simulink model "MMC_phase_centralized_HAAS_20260927"  (R2024b)
settings: Solver=FixedStepDiscrete  StartTime=t_init_sim  StopTime=sim_time  FixedStep=Ts  RelTol=1e-3
values from neighbouring files (symbols this model uses):
  a = 1    [script_MMC_phase_hackathon_NLM_centralized_HAAS_20260927.m]
  C1low1_active = 1    [script_MMC_phase_hackathon_NLM_centralized_HAAS_20260927.m]
  C2low1_active = 1    [script_MMC_phase_hackathon_NLM_centralized_HAAS_20260927.m]
  C_bus = 4400e-6    (= 0.0044)    [script_MMC_phase_hackathon_NLM_centralized_HAAS_20260927.m]
  C_M_extra = C_m-twist_high_side_C    [script_MMC_phase_hackathon_NLM_centralized_HAAS_20260927.m]
  duty_cycle = 1.0    (= 1)    [script_MMC_phase_hackathon_NLM_centralized_HAAS_20260927.m]
  f0 = 50    [script_MMC_phase_hackathon_NLM_centralized_HAAS_20260927.m]
  feeder_current_lower_rate_limit = -10    [script_MMC_phase_hackathon_NLM_centralized_HAAS_20260927.m]    (also in twist_parameters.m = -500)
  feeder_current_tab = [0.328 0.217 0.162 0.132 0.109 0.094 0.083 0.075 0.068 0.062 0.058 0.054 ... (42 elements, 14x3)]    [feeder_current.mat]
  feeder_current_upper_rate_limit = 0.386/(20e-3)    (= 19.3)    [twist_parameters.m]
  is6VExternallySupplied = true    [script_MMC_phase_hackathon_NLM_centralized_HAAS_20260927.m]
  isFeederJumperOpen = true    [script_MMC_phase_hackathon_NLM_centralized_HAAS_20260927.m]
  L_arm = 30e-3    (= 0.03)    [script_MMC_phase_hackathon_NLM_centralized_HAAS_20260927.m]
  m = 1    [script_MMC_phase_hackathon_NLM_centralized_HAAS_20260927.m]
  N = 5    [script_MMC_phase_hackathon_NLM_centralized_HAAS_20260927.m]
  power_losses = false    [script_MMC_phase_hackathon_NLM_centralized_HAAS_20260927.m]
  R = 15    [script_MMC_phase_hackathon_NLM_centralized_HAAS_20260927.m]
  R_arm = 0.2    [script_MMC_phase_hackathon_NLM_centralized_HAAS_20260927.m]
  source_V = 0    [script_MMC_phase_hackathon_NLM_centralized_HAAS_20260927.m]
  Tcom_sample = round(Tcom / Ts)    [script_MMC_phase_hackathon_NLM_centralized_HAAS_20260927.m]
  time_charge = 0.1    [script_MMC_phase_hackathon_NLM_centralized_HAAS_20260927.m]
  time_decharge = 1.5    [script_MMC_phase_hackathon_NLM_centralized_HAAS_20260927.m]
  Ts = 1e-6    (= 1e-06)    [script_MMC_phase_hackathon_NLM_centralized_HAAS_20260927.m]
  twist_data_acquisition_delay = 50e-9    (= 5e-08)    [script_MMC_phase_hackathon_NLM_centralized_HAAS_20260927.m]    (also in twist_parameters.m)
  twist_data_sampling_period = 1/twist_freq_data_sampling    (= 5e-05)    [script_MMC_phase_hackathon_NLM_centralized_HAAS_20260927.m]    (also in twist_parameters.m)
  twist_dead_time = 200e-9    (= 2e-07)    [twist_parameters.m]
  twist_freq_switching = 200e3    (= 200000)    [twist_parameters.m]
  twist_high_side_adc_R = 1/(1/2e6 + 1/2e6 + 1/(330e3+5.6e3))    (= 251272.836178)    [twist_parameters.m]
  twist_high_side_C = 33e-6*4 + 4.7e-6*12    (= 0.0001884)    [twist_parameters.m]
  twist_high_side_feeder_R = 47e3+4.7e3    (= 51700)    [twist_parameters.m]
  twist_high_side_rC = 0.1    [twist_parameters.m]
  twist_low_side_adc_R = 150e3+470    (= 150470)    [twist_parameters.m]
  twist_low_side_C_ceramic = 3*4.7e-6    (= 1.41e-05)    [twist_parameters.m]
  twist_low_side_C_electrolytic = 47e-6    (= 4.7e-05)    [twist_parameters.m]
  twist_low_side_L = 33e-6    (= 3.3e-05)    [twist_parameters.m]
  twist_low_side_rC = 700e-3    (= 0.7)    [twist_parameters.m]
  twist_low_side_rL = 20e-3    (= 0.02)    [twist_parameters.m]
  twist_R_VCC = (tau_VCC/twist_high_side_C  - twist_high_side_rC)/(1-(tau_VCC/twist_high_side_C - twist_high_side_rC)/R_parallel)    (= 1110.74997822)    [twist_parameters.m]
  VDC = 48    [script_MMC_phase_hackathon_NLM_centralized_HAAS_20260927.m]
undefined symbols (not defined in the file or in its folder): C_SM, feeder_current, gcbh, sps_rtmsupport, twist_low_side_lC
libraries: spsSeriesRLCBranchLib x135, spsTriangleGeneratorLib x60, spsMosfetLib x60, spsCurrentMeasurementLib x43, spsVoltageMeasurementLib x35, spsControlledCurrentSourceLib x30, spsDiodeLib x22, spsIdealSwitchLib x20, spsControlledVoltageSourceLib x1, spsGroundLib x1, spspowerguiLib x1
(part 2 of 22)

== system MMC_phase_centralized_HAAS_20260927/ /Sinus Modulation + Sorting Algorithm/M5 MCU1 ==
  g_u : Inport
  M_number : Inport  Port=2
  CVB_upper : MATLAB Function  TreatAsAtomicUnit=on
  g_unitaire_stack : Outport
  wires:
  g_u/1 -> CVB_upper/1(g)
  M_number/1 -> CVB_upper/2(M_number)
  CVB_upper/1(y) -> g_unitaire_stack/1

== system MMC_phase_centralized_HAAS_20260927/ /Sinus Modulation + Sorting Algorithm/M5 MCU2 ==
  g_u : Inport
  M_number : Inport  Port=2
  CVB_upper : MATLAB Function  TreatAsAtomicUnit=on
  g_unitaire_stack : Outport
  wires:
  g_u/1 -> CVB_upper/1(g)
  M_number/1 -> CVB_upper/2(M_number)
  CVB_upper/1(y) -> g_unitaire_stack/1

== system MMC_phase_centralized_HAAS_20260927/ /Sinus Modulation + Sorting Algorithm/M5 MCU3 ==
  g_u : Inport
  M_number : Inport  Port=2
  CVB_upper : MATLAB Function  TreatAsAtomicUnit=on
  g_unitaire_stack : Outport
  wires:
  g_u/1 -> CVB_upper/1(g)
  M_number/1 -> CVB_upper/2(M_number)
  CVB_upper/1(y) -> g_unitaire_stack/1

== system MMC_phase_centralized_HAAS_20260927/ /Sinus Modulation + Sorting Algorithm/M5 MCU4 ==
  g_u : Inport
  M_number : Inport  Port=2
  CVB_upper : MATLAB Function  TreatAsAtomicUnit=on
  g_unitaire_stack : Outport
  wires:
  g_u/1 -> CVB_upper/1(g)
  M_number/1 -> CVB_upper/2(M_number)
  CVB_upper/1(y) -> g_unitaire_stack/1

== system MMC_phase_centralized_HAAS_20260927/ /Sinus Modulation + Sorting Algorithm/M5 MCU5 ==
  g_u : Inport
  M_number : Inport  Port=2
  CVB_upper : MATLAB Function  TreatAsAtomicUnit=on
  g_unitaire_stack : Outport
  wires:
  g_u/1 -> CVB_upper/1(g)
  M_number/1 -> CVB_upper/2(M_number)
  CVB_upper/1(y) -> g_unitaire_stack/1

== system MMC_phase_centralized_HAAS_20260927/ /Sinus Modulation + Sorting Algorithm/Supervisor MCU ==
  note: NLM
  note: NLM
  note: Modulation reference
  note: Sorting and CVB algorithm - Upper and Lower stacks
  note: NLM modulation
  Vc_U : Inport
  I_U : Inport  Port=2
  Vc_L : Inport  Port=3
  I_L : Inport  Port=4
  Constant : Constant
  Constant1 : Constant  Value=0
  Constant2 : Constant
  Constant3 : Constant  Value=0
  Constant4 : Constant  Value=a*1/2
  Gain : Gain  Gain=N
  Gain1 : Gain  Gain=m*1/2
  Gain2 : Gain  Gain=N
  GreaterThan : RelationalOperator  Operator=~=  OutDataTypeStr=boolean  RndMeth=Simplest  InputSameDT=off
  GreaterThan1 : RelationalOperator  Operator=~=  OutDataTypeStr=boolean  RndMeth=Simplest  InputSameDT=off
  Memory : Memory  InheritSampleTime=on  LinearizeMemory=on  LinearizeAsDelay=on
  Memory1 : Memory  InheritSampleTime=on  LinearizeMemory=on  LinearizeAsDelay=on
  Quantizer : Quantizer  QuantizationInterval=1
  Quantizer1 : Quantizer  QuantizationInterval=1
  Saturation : Saturate  UpperLimit=N  LowerLimit=0
  Saturation1 : Saturate  UpperLimit=N  LowerLimit=0
  Sine Wave : Sin  Frequency=2*pi*f0  SampleTime=Ts
  Sorting_CVB_Lower : Subsystem
      settings: PortSchema="{\"entries\":[{\"content\":{\"sides\":[{\"content\":{\"connectorIds\":[\"In1\",\"In2\",\"In3\"]},\"type\":\"ConnectorPlacement.EquallySpacedRectSide\",\"uuid\":\"25566ff9-210a-4488-8b15-702d65e93a4b\"},{\"content\":{\"connectorIds\":[\"Out1\"],\"side\":\"RIGHT\"},\"type\":\"ConnectorPlacement.EquallySpacedRectSide\",\"uuid\":\"97373fc2-3782-4e65-8804-644d53fa5380\"},{\"content\":{\"connectorIds\":[\"In4\"],\"side\":\"TOP\"},\"type\":\"ConnectorPlacement.EquallySpacedRectSide\",\"uuid\":\"e65d2433-d029-4e4a-b081-22e9ded4f272\"}]},\"type\":\"ConnectorPlacement.EquallySpacedConnector\",\"uuid\":\"235c80e7-78ad-4e69-a231-ec76d675b4ae\"}],\"packageUris\":[\"http://schema.mathworks.com/mf0/Connector/R2020b\"],\"version\":\"1.0\"}"
  Sorting_CVB_Upper : Subsystem
      settings: PortSchema="{\"entries\":[{\"content\":{\"sides\":[{\"content\":{\"connectorIds\":[\"In1\",\"In2\",\"In3\"]},\"type\":\"ConnectorPlacement.EquallySpacedRectSide\",\"uuid\":\"25566ff9-210a-4488-8b15-702d65e93a4b\"},{\"content\":{\"connectorIds\":[\"Out1\"],\"side\":\"RIGHT\"},\"type\":\"ConnectorPlacement.EquallySpacedRectSide\",\"uuid\":\"97373fc2-3782-4e65-8804-644d53fa5380\"},{\"content\":{\"connectorIds\":[\"In4\"],\"side\":\"TOP\"},\"type\":\"ConnectorPlacement.EquallySpacedRectSide\",\"uuid\":\"e65d2433-d029-4e4a-b081-22e9ded4f272\"}]},\"type\":\"ConnectorPlacement.EquallySpacedConnector\",\"uuid\":\"235c80e7-78ad-4e69-a231-ec76d675b4ae\"}],\"packageUris\":[\"http://schema.mathworks.com/mf0/Connector/R2020b\"],\"version\":\"1.0\"}"
  Sum1 : Sum  Inputs=|+-
  Sum2 : Sum  Inputs=|++
  Switch : Switch  Criteria=u2 > Threshold  SaturateOnIntegerOverflow=off  InputSameDT=off
  Switch1 : Switch  Criteria=u2 > Threshold  SaturateOnIntegerOverflow=off  InputSameDT=off
  gU : Outport
  gL : Outport  Port=2
  tag scope: N_l=global, N_u=global, ml=global, mu=global
  wires:
  Switch/1 -> Sorting_CVB_Upper/4(Pulse)
  Sorting_CVB_Lower/1(g_unitaire_stack) -> gL/1
  Vc_U/1 -> Sorting_CVB_Upper/1(Vc_unitaire_stack)
  Switch1/1 -> Sorting_CVB_Lower/4(Pulse)
  I_U/1 -> Sorting_CVB_Upper/2(i_stack)
  Quantizer1/1 -> Saturation1/1
  Sorting_CVB_Upper/1(g_unitaire_stack) -> gU/1
  Constant/1 -> Switch/1
  Sine Wave/1 -> Gain1/1
  Saturation/1 -> Sorting_CVB_Upper/3(N_on_stack), Memory/1, GreaterThan/1, [N_u]
  Constant1/1 -> Switch/3
  Saturation1/1 -> Memory1/1, GreaterThan1/1, Sorting_CVB_Lower/3(N_on_stack), [N_l]
  Gain2/1 -> Quantizer1/1
  Constant2/1 -> Switch1/1
  Quantizer/1 -> Saturation/1
  Gain/1 -> Quantizer/1
  GreaterThan/1 -> Switch/2
  Sum1/1 -> Gain/1, [mu]
  Memory1/1 -> GreaterThan1/2
  Gain1/1 -> Sum1/2, Sum2/2
  Constant3/1 -> Switch1/3
  Vc_L/1 -> Sorting_CVB_Lower/1(Vc_unitaire_stack)
  Sum2/1 -> [ml], Gain2/1
  GreaterThan1/1 -> Switch1/2
  Constant4/1 -> Sum2/1, Sum1/1
  Memory/1 -> GreaterThan/2
  I_L/1 -> Sorting_CVB_Lower/2(i_stack)

== system MMC_phase_centralized_HAAS_20260927/ /Subsystem/Subsystem ==
  note: MMC electrical circuit connected to the modules hardware block
  note: MMC electrical circuit connected to the modules hardware block
  note: MMC electrical circuit connected to the modules hardware block
  note: MMC electrical circuit connected to the modules hardware block
  note: MMC electrical circuit connected to the modules hardware block
  duty_cycle_M1 : Inport
  block_M1 : Inport  Port=2
  duty_cycle_M2 : Inport  Port=3
  block_M2 : Inport  Port=4
  duty_cycle_M3 : Inport  Port=5
  block_M3 : Inport  Port=6
  duty_cycle_M4 : Inport  Port=7
  block_M4 : Inport  Port=8
  duty_cycle_M5 : Inport  Port=9
  block_M5 : Inport  Port=10
  AC Load{6..10} (5 alike) : spsSeriesRLCBranchLib/Series RLC Branch  LConnTagsString=__new0  RConnTagsString=__new0  BranchType=C  Resistance=R  Inductance=L_arm  SetiL0=off  InitialCurrent=0  Capacitance=C_M_extra  Setx0=on  InitialVoltage=source_V  Measurements=None
  Hardware M1 : Subsystem
  Hardware M2 : Subsystem
  Hardware M3 : Subsystem
  Hardware M4 : Subsystem
  Hardware M5 : Subsystem
  V1low_M1 : PMIOPort  Side=Left
  Low_GND_M5 : PMIOPort  Port=2  Side=Left
  i_mod_M1 : Outport
  v_cap_M1 : Outport  Port=2
  v_cap_M2 : Outport  Port=3
  v_cap_M3 : Outport  Port=4
  v_cap_M4 : Outport  Port=5
  v_cap_M5 : Outport  Port=6
  wires:
  Hardware M1/1(v_cap) -> v_cap_M1/1
  duty_cycle_M1/1 -> Hardware M1/1(duty_cycle)
  duty_cycle_M2/1 -> Hardware M2/1(duty_cycle)
  block_M5/1 -> Hardware M5/2(block)
  Hardware M3/1(v_cap) -> v_cap_M3/1
  block_M1/1 -> Hardware M1/2(block)
  Hardware M1/2(i_mod) -> i_mod_M1/1
  duty_cycle_M4/1 -> Hardware M4/1(duty_cycle)
  block_M2/1 -> Hardware M2/2(block)
  Hardware M5/1(v_cap) -> v_cap_M5/1
  Hardware M2/1(v_cap) -> v_cap_M2/1
  duty_cycle_M3/1 -> Hardware M3/1(duty_cycle)
  duty_cycle_M5/1 -> Hardware M5/1(duty_cycle)
  block_M4/1 -> Hardware M4/2(block)
  block_M3/1 -> Hardware M3/2(block)
  Hardware M4/1(v_cap) -> v_cap_M4/1
  connections:
  Hardware M5/RConn2 -- AC Load10/RConn1
  AC Load6/LConn1 -- Hardware M1/RConn1
  Hardware M1/LConn2 -- Hardware M2/LConn1
  Hardware M3/LConn2 -- Hardware M4/LConn1
  Hardware M5/RConn1 -- AC Load10/LConn1
  AC Load6/RConn1 -- Hardware M1/RConn2
  Hardware M2/RConn2 -- AC Load7/RConn1
  Hardware M2/LConn2 -- Hardware M3/LConn1
  Hardware M2/RConn1 -- AC Load7/LConn1
  Hardware M3/RConn1 -- AC Load8/LConn1
  Hardware M3/RConn2 -- AC Load8/RConn1
  Hardware M4/RConn2 -- AC Load9/RConn1
  Hardware M4/RConn1 -- AC Load9/LConn1
  Hardware M4/LConn2 -- Hardware M5/LConn1
  V1low_M1/RConn1 -- Hardware M1/LConn1
  Low_GND_M5/RConn1 -- Hardware M5/LConn2

== system MMC_phase_centralized_HAAS_20260927/ /Subsystem/Subsystem1 ==
  note: MMC electrical circuit connected to the modules hardware block
  note: MMC electrical circuit connected to the modules hardware block
  note: MMC electrical circuit connected to the modules hardware block
  note: MMC electrical circuit connected to the modules hardware block
  note: MMC electrical circuit connected to the modules hardware block
  duty_cycle_M1 : Inport
  block_M1 : Inport  Port=2
  duty_cycle_M2 : Inport  Port=3
  block_M2 : Inport  Port=4
  duty_cycle_M3 : Inport  Port=5
  block_M3 : Inport  Port=6
  duty_cycle_M4 : Inport  Port=7
  block_M4 : Inport  Port=8
  duty_cycle_M5 : Inport  Port=9
  block_M5 : Inport  Port=10
  AC Load{6..10} (5 alike) : spsSeriesRLCBranchLib/Series RLC Branch  LConnTagsString=__new0  RConnTagsString=__new0  BranchType=C  Resistance=R  Inductance=L_arm  SetiL0=off  InitialCurrent=0  Capacitance=C_M_extra  Setx0=on  InitialVoltage=source_V  Measurements=None
  Hardware M1 : Subsystem
  Hardware M2 : Subsystem
  Hardware M3 : Subsystem
  Hardware M4 : Subsystem
  Hardware M5 : Subsystem
  V1low_M1 : PMIOPort  Side=Left
  Low_GND_M5 : PMIOPort  Port=2  Side=Left
  i_mod_M1 : Outport
  v_cap_M1 : Outport  Port=2
  v_cap_M2 : Outport  Port=3
  v_cap_M3 : Outport  Port=4
  v_cap_M4 : Outport  Port=5
  v_cap_M5 : Outport  Port=6
  wires:
  Hardware M1/1(v_cap) -> v_cap_M1/1
  duty_cycle_M1/1 -> Hardware M1/1(duty_cycle)
  duty_cycle_M2/1 -> Hardware M2/1(duty_cycle)
  block_M5/1 -> Hardware M5/2(block)
  Hardware M3/1(v_cap) -> v_cap_M3/1
  block_M1/1 -> Hardware M1/2(block)
  Hardware M1/2(i_mod) -> i_mod_M1/1
  duty_cycle_M4/1 -> Hardware M4/1(duty_cycle)
  block_M2/1 -> Hardware M2/2(block)
  Hardware M5/1(v_cap) -> v_cap_M5/1
  Hardware M2/1(v_cap) -> v_cap_M2/1
  duty_cycle_M3/1 -> Hardware M3/1(duty_cycle)
  duty_cycle_M5/1 -> Hardware M5/1(duty_cycle)
  block_M4/1 -> Hardware M4/2(block)
  block_M3/1 -> Hardware M3/2(block)
  Hardware M4/1(v_cap) -> v_cap_M4/1
  connections:
  Hardware M5/RConn2 -- AC Load10/RConn1
  AC Load6/LConn1 -- Hardware M1/RConn1
  Hardware M1/LConn2 -- Hardware M2/LConn1
  Hardware M3/LConn2 -- Hardware M4/LConn1
  Hardware M5/RConn1 -- AC Load10/LConn1
  AC Load6/RConn1 -- Hardware M1/RConn2
  Hardware M2/RConn2 -- AC Load7/RConn1
  Hardware M2/LConn2 -- Hardware M3/LConn1
  Hardware M2/RConn1 -- AC Load7/LConn1
  Hardware M3/RConn1 -- AC Load8/LConn1
  Hardware M3/RConn2 -- AC Load8/RConn1
  Hardware M4/RConn2 -- AC Load9/RConn1
  Hardware M4/RConn1 -- AC Load9/LConn1
  Hardware M4/LConn2 -- Hardware M5/LConn1
  V1low_M1/RConn1 -- Hardware M1/LConn1
  Low_GND_M5/RConn1 -- Hardware M5/LConn2

== system MMC_phase_centralized_HAAS_20260927/ /Communication_subsystem/Lower_arm/M1_Comm ==
  TX_variables : Inport
  sync : Inport  Port=2
  RX_signal : Inport  Port=3
  Data Type Conversion : DataTypeConversion  OutDataTypeStr=single  SaturateOnIntegerOverflow=off  RndMeth=Floor
  Delay : Delay  DelayLength=Tcom_sample
  Snapshot : MATLAB Function  TreatAsAtomicUnit=on
  TxFormatter : MATLAB Function  TreatAsAtomicUnit=on
  node_id : Constant  Value=6
  TX_signal : Outport
  RX_Variables : Outport  Port=2
  wires:
  TX_variables/1 -> Data Type Conversion/1
  RX_signal/1 -> Snapshot/1(rx_signal), TxFormatter/3(rx_signal)
  TxFormatter/1(tx_data) -> Delay/1
  Data Type Conversion/1 -> TxFormatter/1(tx_variables)
  Snapshot/1(rx_variables) -> RX_Variables/1
  sync/1 -> Snapshot/3(sync), TxFormatter/2(sync)
  node_id/1 -> TxFormatter/4(node_id)
  Delay/1 -> TX_signal/1

== system MMC_phase_centralized_HAAS_20260927/ /Communication_subsystem/Lower_arm/M2_Comm ==
  TX_variables : Inport
  sync : Inport  Port=2
  RX_signal : Inport  Port=3
  Data Type Conversion : DataTypeConversion  OutDataTypeStr=single  SaturateOnIntegerOverflow=off  RndMeth=Floor
  Delay : Delay  DelayLength=Tcom_sample
  Snapshot : MATLAB Function  TreatAsAtomicUnit=on
  TxFormatter : MATLAB Function  TreatAsAtomicUnit=on
  node_id : Constant  Value=7
  TX_signal : Outport
  RX_Variables : Outport  Port=2
  wires:
  TX_variables/1 -> Data Type Conversion/1
  RX_signal/1 -> Snapshot/1(rx_signal), TxFormatter/3(rx_signal)
  TxFormatter/1(tx_data) -> Delay/1
  Data Type Conversion/1 -> TxFormatter/1(tx_variables)
  Snapshot/1(rx_variables) -> RX_Variables/1
  sync/1 -> Snapshot/3(sync), TxFormatter/2(sync)
  node_id/1 -> TxFormatter/4(node_id)
  Delay/1 -> TX_signal/1

== system MMC_phase_centralized_HAAS_20260927/ /Communication_subsystem/Lower_arm/M3_Comm ==
  TX_variables : Inport
  sync : Inport  Port=2
  RX_signal : Inport  Port=3
  Data Type Conversion : DataTypeConversion  OutDataTypeStr=single  SaturateOnIntegerOverflow=off  RndMeth=Floor
  Delay : Delay  DelayLength=Tcom_sample
  Snapshot : MATLAB Function  TreatAsAtomicUnit=on
  TxFormatter : MATLAB Function  TreatAsAtomicUnit=on
  node_id : Constant  Value=8
  TX_signal : Outport
  RX_Variables : Outport  Port=2
  wires:
  TX_variables/1 -> Data Type Conversion/1
  RX_signal/1 -> Snapshot/1(rx_signal), TxFormatter/3(rx_signal)
  TxFormatter/1(tx_data) -> Delay/1
  Data Type Conversion/1 -> TxFormatter/1(tx_variables)
  Snapshot/1(rx_variables) -> RX_Variables/1
  sync/1 -> Snapshot/3(sync), TxFormatter/2(sync)
  node_id/1 -> TxFormatter/4(node_id)
  Delay/1 -> TX_signal/1

== system MMC_phase_centralized_HAAS_20260927/ /Communication_subsystem/Lower_arm/M4_Comm ==
  TX_variables : Inport
  sync : Inport  Port=2
  RX_signal : Inport  Port=3
  Data Type Conversion : DataTypeConversion  OutDataTypeStr=single  SaturateOnIntegerOverflow=off  RndMeth=Floor
  Delay : Delay  DelayLength=Tcom_sample
  Snapshot : MATLAB Function  TreatAsAtomicUnit=on
  TxFormatter : MATLAB Function  TreatAsAtomicUnit=on
  node_id : Constant  Value=9
  TX_signal : Outport
  RX_Variables : Outport  Port=2
  wires:
  TX_variables/1 -> Data Type Conversion/1
  RX_signal/1 -> Snapshot/1(rx_signal), TxFormatter/3(rx_signal)
  TxFormatter/1(tx_data) -> Delay/1
  Data Type Conversion/1 -> TxFormatter/1(tx_variables)
  Snapshot/1(rx_variables) -> RX_Variables/1
  sync/1 -> Snapshot/3(sync), TxFormatter/2(sync)
  node_id/1 -> TxFormatter/4(node_id)
  Delay/1 -> TX_signal/1

== system MMC_phase_centralized_HAAS_20260927/ /Communication_subsystem/Lower_arm/M5_Comm ==
  TX_variables : Inport
  sync : Inport  Port=2
  RX_signal : Inport  Port=3
  Data Type Conversion : DataTypeConversion  OutDataTypeStr=single  SaturateOnIntegerOverflow=off  RndMeth=Floor
  Delay : Delay  DelayLength=Tcom_sample
  Snapshot : MATLAB Function  TreatAsAtomicUnit=on
  TxFormatter : MATLAB Function  TreatAsAtomicUnit=on
  node_id : Constant  Value=10
  TX_signal : Outport
  RX_Variables : Outport  Port=2
  wires:
  TX_variables/1 -> Data Type Conversion/1
  RX_signal/1 -> Snapshot/1(rx_signal), TxFormatter/3(rx_signal)
  TxFormatter/1(tx_data) -> Delay/1
  Data Type Conversion/1 -> TxFormatter/1(tx_variables)
  Snapshot/1(rx_variables) -> RX_Variables/1
  sync/1 -> Snapshot/3(sync), TxFormatter/2(sync)
  node_id/1 -> TxFormatter/4(node_id)
  Delay/1 -> TX_signal/1

== system MMC_phase_centralized_HAAS_20260927/ /Communication_subsystem/Upper_arm/M1_Comm ==
  TX_variables : Inport
  sync : Inport  Port=2
  RX_signal : Inport  Port=3
  Data Type Conversion : DataTypeConversion  OutDataTypeStr=single  SaturateOnIntegerOverflow=off  RndMeth=Floor
  Delay : Delay  DelayLength=Tcom_sample
  Delay1 : Delay  DelayLength=1
  Delay2 : Delay  DelayLength=1
  Scope : Scope  NumInputPorts=6
  Scope1 : Scope  NumInputPorts=2
  Snapshot : MATLAB Function  TreatAsAtomicUnit=on
  TxFormatter : MATLAB Function  TreatAsAtomicUnit=on
  node_id : Constant
  TX_signal : Outport
  RX_Variables : Outport  Port=2
  wires:
  TX_variables/1 -> Data Type Conversion/1
  TxFormatter/1(tx_data) -> Delay/1
  Delay/1 -> TX_signal/1
  sync/1 -> Snapshot/3(sync), Scope1/1, TxFormatter/2(sync)  "Ctrl_task"
  RX_signal/1 -> Snapshot/1(rx_signal), TxFormatter/3(rx_signal)
  Snapshot/1(rx_variables) -> RX_Variables/1
  Data Type Conversion/1 -> TxFormatter/1(tx_variables)
  node_id/1 -> TxFormatter/4(node_id)
  TxFormatter/2(tx_fire) -> Scope/1
  TxFormatter/3(tx_busy) -> Scope/2
  TxFormatter/5(rx_count_dbg) -> Scope/4
  TxFormatter/6(rx_id_dbg) -> Scope1/2, Scope/5  "1 -> 2 data"
  TxFormatter/7(overrun) -> Scope/6
  TxFormatter/8(local_frame_snapshot) -> Delay1/1
  Delay1/1 -> Snapshot/2(local_frame_snapshot)
  TxFormatter/4(round_done) -> Scope/3, Delay2/1
  Delay2/1 -> Snapshot/4(round_done)

== system MMC_phase_centralized_HAAS_20260927/ /Communication_subsystem/Upper_arm/M2_Comm ==
  TX_variables : Inport
  sync : Inport  Port=2
  RX_signal : Inport  Port=3
  Data Type Conversion : DataTypeConversion  OutDataTypeStr=single  SaturateOnIntegerOverflow=off  RndMeth=Floor
  Delay : Delay  DelayLength=Tcom_sample
  Delay1 : Delay  DelayLength=1
  Scope : Scope  NumInputPorts=6
  Snapshot : MATLAB Function  TreatAsAtomicUnit=on
  TxFormatter : MATLAB Function  TreatAsAtomicUnit=on
  node_id : Constant  Value=2
  TX_signal : Outport
  RX_Variables : Outport  Port=2
  wires:
  TxFormatter/2(tx_fire) -> Scope/1
  TxFormatter/3(tx_busy) -> Scope/2
  TxFormatter/8(local_frame_snapshot) -> Delay1/1
  TxFormatter/7(overrun) -> Scope/6
  TX_variables/1 -> Data Type Conversion/1
  Delay/1 -> TX_signal/1
  TxFormatter/4(round_done) -> Scope/3
  Snapshot/1(rx_variables) -> RX_Variables/1
  TxFormatter/1(tx_data) -> Delay/1
  Delay1/1 -> Snapshot/2(local_frame_snapshot)
  Data Type Conversion/1 -> TxFormatter/1(tx_variables)
  sync/1 -> Snapshot/3(sync), TxFormatter/2(sync)
  node_id/1 -> TxFormatter/4(node_id)
  TxFormatter/6(rx_id_dbg) -> Scope/5
  RX_signal/1 -> Snapshot/1(rx_signal), TxFormatter/3(rx_signal)
  TxFormatter/5(rx_count_dbg) -> Scope/4

== system MMC_phase_centralized_HAAS_20260927/ /Communication_subsystem/Upper_arm/M3_Comm ==
  TX_variables : Inport
  sync : Inport  Port=2
  RX_signal : Inport  Port=3
  Data Type Conversion : DataTypeConversion  OutDataTypeStr=single  SaturateOnIntegerOverflow=off  RndMeth=Floor
  Delay : Delay  DelayLength=Tcom_sample
  Delay1 : Delay  DelayLength=1
  Scope : Scope  NumInputPorts=6
  Snapshot : MATLAB Function  TreatAsAtomicUnit=on
  TxFormatter : MATLAB Function  TreatAsAtomicUnit=on
  node_id : Constant  Value=3
  TX_signal : Outport
  RX_Variables : Outport  Port=2
  wires:
  TxFormatter/2(tx_fire) -> Scope/1
  TxFormatter/3(tx_busy) -> Scope/2
  TxFormatter/8(local_frame_snapshot) -> Delay1/1
  TxFormatter/7(overrun) -> Scope/6
  TX_variables/1 -> Data Type Conversion/1
  Delay/1 -> TX_signal/1
  TxFormatter/4(round_done) -> Scope/3
  Snapshot/1(rx_variables) -> RX_Variables/1
  TxFormatter/1(tx_data) -> Delay/1
  Delay1/1 -> Snapshot/2(local_frame_snapshot)
  Data Type Conversion/1 -> TxFormatter/1(tx_variables)
  sync/1 -> Snapshot/3(sync), TxFormatter/2(sync)
  node_id/1 -> TxFormatter/4(node_id)
  TxFormatter/6(rx_id_dbg) -> Scope/5
  RX_signal/1 -> Snapshot/1(rx_signal), TxFormatter/3(rx_signal)
  TxFormatter/5(rx_count_dbg) -> Scope/4

== system MMC_phase_centralized_HAAS_20260927/ /Communication_subsystem/Upper_arm/M4_Comm ==
  TX_variables : Inport
  sync : Inport  Port=2
  RX_signal : Inport  Port=3
  Data Type Conversion : DataTypeConversion  OutDataTypeStr=single  SaturateOnIntegerOverflow=off  RndMeth=Floor
  Delay : Delay  DelayLength=Tcom_sample
  Delay1 : Delay  DelayLength=1
  Scope : Scope  NumInputPorts=6
  Snapshot : MATLAB Function  TreatAsAtomicUnit=on
  TxFormatter : MATLAB Function  TreatAsAtomicUnit=on
  node_id : Constant  Value=4
  TX_signal : Outport
  RX_Variables : Outport  Port=2
  wires:
  TxFormatter/2(tx_fire) -> Scope/1
  TxFormatter/3(tx_busy) -> Scope/2
  TxFormatter/8(local_frame_snapshot) -> Delay1/1
  TxFormatter/7(overrun) -> Scope/6
  TX_variables/1 -> Data Type Conversion/1
  Delay/1 -> TX_signal/1
  TxFormatter/4(round_done) -> Scope/3
  Snapshot/1(rx_variables) -> RX_Variables/1
  TxFormatter/1(tx_data) -> Delay/1
  Delay1/1 -> Snapshot/2(local_frame_snapshot)
  Data Type Conversion/1 -> TxFormatter/1(tx_variables)
  sync/1 -> Snapshot/3(sync), TxFormatter/2(sync)
  node_id/1 -> TxFormatter/4(node_id)
  TxFormatter/6(rx_id_dbg) -> Scope/5
  RX_signal/1 -> Snapshot/1(rx_signal), TxFormatter/3(rx_signal)
  TxFormatter/5(rx_count_dbg) -> Scope/4

== system MMC_phase_centralized_HAAS_20260927/ /Communication_subsystem/Upper_arm/M5_Comm ==
  TX_variables : Inport
  sync : Inport  Port=2
  RX_signal : Inport  Port=3
  Data Type Conversion : DataTypeConversion  OutDataTypeStr=single  SaturateOnIntegerOverflow=off  RndMeth=Floor
  Delay : Delay  DelayLength=Tcom_sample
  Snapshot : MATLAB Function  TreatAsAtomicUnit=on
  TxFormatter : MATLAB Function  TreatAsAtomicUnit=on
  node_id : Constant  Value=5
  TX_signal : Outport
  RX_Variables : Outport  Port=2
  wires:
  TX_variables/1 -> Data Type Conversion/1
  RX_signal/1 -> Snapshot/1(rx_signal), TxFormatter/3(rx_signal)
  TxFormatter/1(tx_data) -> Delay/1
  Data Type Conversion/1 -> TxFormatter/1(tx_variables)
  Snapshot/1(rx_variables) -> RX_Variables/1
  sync/1 -> Snapshot/3(sync), TxFormatter/2(sync)
  node_id/1 -> TxFormatter/4(node_id)
  Delay/1 -> TX_signal/1

== system MMC_phase_centralized_HAAS_20260927/ /Sinus Modulation + Sorting Algorithm/Supervisor MCU/Sorting_CVB_Lower ==
  Vc_unitaire_stack : Inport
  i_stack : Inport  Port=2
  N_on_stack : Inport  Port=3
  Pulse : Inport  Port=4
  CVB : MATLAB Function  TreatAsAtomicUnit=on
  Constant : Constant  Value=duty_cycle
  Scope : Scope  NumInputPorts=5
  Sorting : Subsystem
  g_unitaire_stack : Outport
  wires:
  Vc_unitaire_stack/1 -> Sorting/1(Vc_u), Scope/1
  Sorting/1(Ordre_u) -> CVB/1(ordre)
  N_on_stack/1 -> Scope/4, CVB/3(N_on)
  i_stack/1 -> Scope/2, Sorting/2(i_u)
  Sorting/2(Sens_u) -> CVB/2(sens)
  Pulse/1 -> Scope/5, Sorting/Enable
  CVB/1(y) -> Scope/3, g_unitaire_stack/1
  Constant/1 -> CVB/4(duty_cycle)

== system MMC_phase_centralized_HAAS_20260927/ /Sinus Modulation + Sorting Algorithm/Supervisor MCU/Sorting_CVB_Upper ==
  Vc_unitaire_stack : Inport
  i_stack : Inport  Port=2
  N_on_stack : Inport  Port=3
  Pulse : Inport  Port=4
  CVB : MATLAB Function  TreatAsAtomicUnit=on
  Constant : Constant  Value=duty_cycle
  Scope : Scope  NumInputPorts=5
  Sorting : Subsystem
  g_unitaire_stack : Outport
  wires:
  Vc_unitaire_stack/1 -> Sorting/1(Vc_u), Scope/1
  Sorting/1(Ordre_u) -> CVB/1(ordre)
  N_on_stack/1 -> Scope/4, CVB/3(N_on)
  i_stack/1 -> Scope/2, Sorting/2(i_u)
  Sorting/2(Sens_u) -> CVB/2(sens)
  Pulse/1 -> Scope/5, Sorting/Enable
  CVB/1(y) -> Scope/3, g_unitaire_stack/1
  Constant/1 -> CVB/4(duty_cycle)

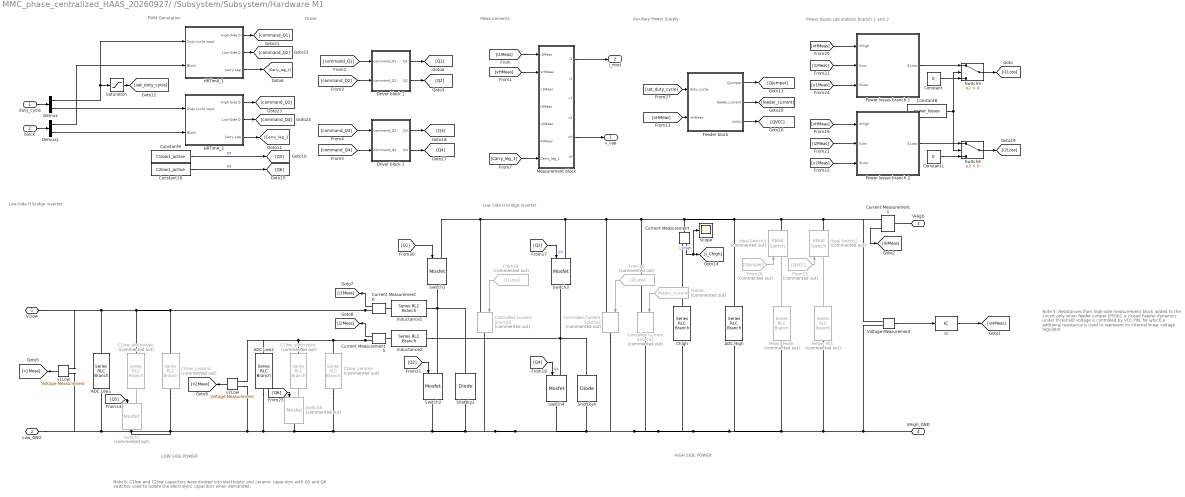
== system MMC_phase_centralized_HAAS_20260927/ /Subsystem/Subsystem/Hardware M1 ==
  note: Low Side H bridge inverter
  note: PWM Generation
  note: Auxiliary Power Supply
  note: LOW SIDE POWER
  note: Low-Side H bridge inverter
  note: Power losses calculations branch 1 and 2
  note: Note 6:
      | C1low and C2low capacitors were divided into electrolytic and ceramic capacitors with Q5 and Q6 switches used to isolate the electrolytic capacitors when demanded.
  note: HIGH SIDE POWER
  note: Measurements
  note: Note 5:
      |
      | Resistances from high-side measurement block added to the circuit only when feeder jumper JP5001 is closed
      |
      | Feeder dynamics under threshold voltage is controlled by VCC PIN, for which a addtional resistance is used to represent its internal linear voltage regulator
  note: Driver
  duty_cycle : Inport
  block : Inport  Port=2
  ADC High : spsSeriesRLCBranchLib/Series RLC Branch  LConnTagsString=__new0  RConnTagsString=__new0  BranchType=R  Resistance=twist_high_side_adc_R  Inductance=twist_low_side_L  SetiL0=off  InitialCurrent=0  Capacitance=1e-6  Setx0=off  InitialVoltage=0  Measurements=None
  ADC Low1 : spsSeriesRLCBranchLib/Series RLC Branch  LConnTagsString=__new0  RConnTagsString=__new0  BranchType=R  Resistance=twist_low_side_adc_R  Inductance=twist_low_side_L  SetiL0=off  InitialCurrent=0  Capacitance=1e-6  Setx0=off  InitialVoltage=0  Measurements=Branch voltage
  ADC Low2 : spsSeriesRLCBranchLib/Series RLC Branch  LConnTagsString=__new0  RConnTagsString=__new0  BranchType=R  Resistance=twist_low_side_adc_R  Inductance=twist_low_side_L  SetiL0=off  InitialCurrent=0  Capacitance=1e-6  Setx0=off  InitialVoltage=0  Measurements=Branch voltage
  C1low_ceramic : spsSeriesRLCBranchLib/Series RLC Branch  Commented=on  LConnTagsString=__new0  RConnTagsString=__new0  BranchType=C  Resistance=twist_low_side_rC  Inductance=1e-3  SetiL0=off  InitialCurrent=0  Capacitance=twist_low_side_C_ceramic  Setx0=off  InitialVoltage=source_V  Measurements=None
  C1low_electrolytic : spsSeriesRLCBranchLib/Series RLC Branch  Commented=on  LConnTagsString=__new0  RConnTagsString=__new0  BranchType=RC  Resistance=twist_low_side_rC  Inductance=twist_low_side_lC  SetiL0=off  InitialCurrent=0  Capacitance=twist_low_side_C_electrolytic  Setx0=off  InitialVoltage=source_V  Measurements=None
  C2low_ceramic : spsSeriesRLCBranchLib/Series RLC Branch  Commented=on  LConnTagsString=__new0  RConnTagsString=__new0  BranchType=C  Resistance=twist_low_side_rC  Inductance=1e-3  SetiL0=off  InitialCurrent=0  Capacitance=twist_low_side_C_ceramic  Setx0=off  InitialVoltage=source_V  Measurements=None
  C2low_electrolytic : spsSeriesRLCBranchLib/Series RLC Branch  Commented=on  LConnTagsString=__new0  RConnTagsString=__new0  BranchType=RC  Resistance=twist_low_side_rC  Inductance=twist_low_side_lC  SetiL0=off  InitialCurrent=0  Capacitance=twist_low_side_C_electrolytic  Setx0=off  InitialVoltage=source_V  Measurements=None
  Chigh : spsSeriesRLCBranchLib/Series RLC Branch  LConnTagsString=__new0  RConnTagsString=__new0  BranchType=RC  Resistance=twist_high_side_rC  Inductance=1e-3  SetiL0=off  InitialCurrent=0  Capacitance=twist_high_side_C  Setx0=on  InitialVoltage=source_V  Measurements=None
  Constant : Constant  Value=0
  Constant1 : Constant  Value=0
  Constant10 : Constant  Value=C2low1_active
  Constant8 : Constant  Value=power_losses
  Constant9 : Constant  Value=C1low1_active
  Controlled Current Source1 : spsControlledCurrentSourceLib/Controlled Current Source  Commented=on  Initialize=on  Source_Type=AC  Amplitude=0  Phase=0  Frequency=0  Measurements=None
  Controlled Current Source2 : spsControlledCurrentSourceLib/Controlled Current Source  Commented=on  Initialize=on  Source_Type=AC  Amplitude=0  Phase=0  Frequency=0  Measurements=None
  Controlled Current Source3 : spsControlledCurrentSourceLib/Controlled Current Source  Commented=on  Initialize=on  Source_Type=AC  Amplitude=0  Phase=0  Frequency=0  Measurements=None
  Current Measurement{,1,5..6} (4 alike) : spsCurrentMeasurementLib/Current Measurement  PhasorSimulation=off  OutputType=Complex  PSBequivalent=0
  Demux : Demux  Outputs=2
  Demux1 : Demux  Outputs=2
  Driver block 1 : Subsystem
  Driver block 2 : Subsystem
  Feeder block : Subsystem
  From15 : From  Commented=on  GotoTag=QVCC
  From16 : From  Commented=on  GotoTag=i2Loss
  From26 : From  Commented=on  GotoTag=Qjumper
  From28 : From  Commented=on  GotoTag=i1Loss
  From6 : From  Commented=on  GotoTag=feeder_current
  HRTimA_1 : Subsystem
  HRTimA_2 : Subsystem
  IC : InitialCondition  Value=source_V
  Ideal Switch1 : spsIdealSwitchLib/Ideal Switch  Commented=on  Ron=0.001  Lon=0  IC=0  Rs=1e5  Cs=inf  Measurements=on
  Ideal Switch2 : spsIdealSwitchLib/Ideal Switch  Commented=on  Ron=0.001  Lon=0  IC=0  Rs=1e5  Cs=inf  Measurements=on
  Inductance1 : spsSeriesRLCBranchLib/Series RLC Branch  LConnTagsString=__new0  RConnTagsString=__new0  BranchType=RL  Resistance=twist_low_side_rL  Inductance=twist_low_side_L  SetiL0=off  InitialCurrent=0  Capacitance=1e-6  Setx0=off  InitialVoltage=0  Measurements=None
  Inductance2 : spsSeriesRLCBranchLib/Series RLC Branch  LConnTagsString=__new0  RConnTagsString=__new0  BranchType=RL  Resistance=twist_low_side_rL  Inductance=twist_low_side_L  SetiL0=off  InitialCurrent=0  Capacitance=1e-6  Setx0=off  InitialVoltage=0  Measurements=None
  Meas Feeder : spsSeriesRLCBranchLib/Series RLC Branch  Commented=on  LConnTagsString=__new0  RConnTagsString=__new0  BranchType=R  Resistance=twist_high_side_feeder_R  Inductance=twist_low_side_L  SetiL0=off  InitialCurrent=0  Capacitance=1e-6  Setx0=off  InitialVoltage=0  Measurements=None
  Measurement block : Subsystem
  Power losses branch 1 : Subsystem
  Power losses branch 2 : Subsystem
  Saturation : Saturate  UpperLimit=1  LowerLimit=0
  Scope : Scope
  Shottky2 : spsDiodeLib/Diode  Ron=twist_shottky_Ron  Lon=0  Vf=twist_shottky_Vf  IC=0  UseSnubber=0  Rs=twist_shottky_Rs  Cs=twist_shottky_Cs  Measurements=off
  Shottky4 : spsDiodeLib/Diode  Ron=twist_shottky_Ron  Lon=0  Vf=twist_shottky_Vf  IC=0  UseSnubber=0  Rs=twist_shottky_Rs  Cs=twist_shottky_Cs  Measurements=off
  Switch{1..4} (4 alike) : spsMosfetLib/Mosfet  Ron=twist_FET_Ron  Lon=0  Rd=twist_FET_Rd  Vfd=twist_FET_Vf  IC=0  Rs=twist_FET_Rs  Cs=twist_FET_Cs  Measurements=off
  Switch5 : Switch  Criteria=u2 > Threshold  SaturateOnIntegerOverflow=off  InputSameDT=off
  Switch6 : Switch  Criteria=u2 > Threshold  SaturateOnIntegerOverflow=off  InputSameDT=off
  Switch7 : spsMosfetLib/Mosfet  Commented=on  Ron=twist_FET_Clow_Ron  Lon=0  Rd=twist_FET_Clow_Ron  Vfd=0  IC=0  Rs=twist_FET_Rs  Cs=twist_FET_Cs  Measurements=off
  Switch8 : spsMosfetLib/Mosfet  Commented=on  Ron=twist_FET_Clow_Ron  Lon=0  Rd=twist_FET_Clow_Ron  Vfd=0  IC=0  Rs=twist_FET_Rs  Cs=twist_FET_Cs  Measurements=off
  Voltage Measurement : spsVoltageMeasurementLib/Voltage Measurement  PhasorSimulation=off  OutputType=Complex  PSBequivalent=0
  feeder VCC : spsSeriesRLCBranchLib/Series RLC Branch  Commented=on  LConnTagsString=__new0  RConnTagsString=__new0  BranchType=R  Resistance=twist_R_VCC  Inductance=twist_low_side_L  SetiL0=off  InitialCurrent=0  Capacitance=1e-6  Setx0=off  InitialVoltage=0  Measurements=None
  v1Low : spsVoltageMeasurementLib/Voltage Measurement  PhasorSimulation=off  OutputType=Complex  PSBequivalent=0
  v2Low : spsVoltageMeasurementLib/Voltage Measurement  PhasorSimulation=off  OutputType=Complex  PSBequivalent=0
  V1low : PMIOPort  Side=Left
  Low_GND : PMIOPort  Port=2  Side=Left
  VHigh : PMIOPort  Port=3  Side=Right
  VHigh_GND : PMIOPort  Port=4  Side=Right
  v_cap : Outport
  i_mod : Outport  Port=2
  wires:
  Constant8/1 -> Switch5/2, Switch6/2
  Constant9/1 -> [Q5]  "Q5"
  Constant1/1 -> Switch6/3
  v1Low/1 -> [v1Meas]
  Power losses branch 1/1(i1Loss) -> Switch5/1
  Constant/1 -> Switch5/3
  [Q1] -> Switch1/1
  [Q3] -> Switch3/1  "Q3"
  Voltage Measurement/1 -> IC/1
  Constant10/1 -> [Q6]  "Q6"
  [v1Meas] -> Power losses branch 1/3(VLow)
  [i2Meas] -> Power losses branch 2/2(ILow)
  Switch5/1 -> [i1Loss]
  HRTimA_2/3(Carry Leg) -> [Carry_leg_2]
  Current Measurement1/1 -> [iHMeas]
  v2Low/1 -> [v2Meas]
  HRTimA_1/3(Carry Leg) -> [Carry_leg_1]
  [vHMeas] -> Power losses branch 1/1(VHigh)
  IC/1 -> [vHMeas]
  From28/1 -> Controlled Current Source3/1
  Current Measurement/1 -> Scope/1, [i_Chigh]  "i_Chigh"
  Switch6/1 -> [i2Loss]
  Current Measurement5/1 -> [i2Meas]
  From26/1 -> Ideal Switch1/1
  [i1Meas] -> Power losses branch 1/2(ILow)
  From15/1 -> Ideal Switch2/1
  [Q5] -> Switch7/1
  [Q6] -> Switch8/1
  [Q4] -> Switch4/1  "Q4"
  [Q2] -> Switch2/1
  From6/1 -> Controlled Current Source1/1
  [vHMeas] -> Power losses branch 2/1(VHigh)
  From16/1 -> Controlled Current Source2/1
  [v2Meas] -> Power losses branch 2/3(VLow)
  Current Measurement6/1 -> [i1Meas]
  Power losses branch 2/1(i1Loss) -> Switch6/1
  duty_cycle/1 -> Demux/1
  Demux/1 -> Saturation/1, HRTimA_1/1(Duty cycle input)
  Demux1/1 -> HRTimA_1/2(Block)
  block/1 -> Demux1/1
  Demux1/2 -> HRTimA_2/2(Block)
  Demux/2 -> HRTimA_2/1(Duty cycle input)
  [vHMeas] -> Feeder block/2(vHMeas)
  Saturation/1 -> [sat_duty_cycle]
  [sat_duty_cycle] -> Feeder block/1(duty_cycle)
  Feeder block/1(Qjumper) -> [Qjumper]
  Feeder block/3(QVCC) -> [QVCC]
  Feeder block/2(feeder_current) -> [feeder_current]
  Measurement block/1(i1) -> i_mod/1
  [i1Meas] -> Measurement block/1(i1Meas)
  [vHMeas] -> Measurement block/2(vHMeas)
  Measurement block/5(vH) -> v_cap/1
  HRTimA_1/1(High-Side Q) -> [command_Q1]
  HRTimA_1/2(Low-Side Q) -> [command_Q2]
  HRTimA_2/1(High-Side Q) -> [command_Q3]
  HRTimA_2/2(Low-Side Q) -> [command_Q4]
  [command_Q1] -> Driver block 1/1(command_Q1)
  [command_Q2] -> Driver block 1/2(command_Q2)
  [command_Q3] -> Driver block 2/1(command_Q3)
  [command_Q4] -> Driver block 2/2(command_Q4)
  Driver block 1/1(Q1) -> [Q1]
  Driver block 1/2(Q2) -> [Q2]
  Driver block 2/1(Q3) -> [Q3]
  Driver block 2/2(Q4) -> [Q4]
  [Carry_leg_1] -> Measurement block/7(Carry_leg_1)
  connections:
  Current Measurement6/RConn1 -- v1Low/LConn1 -- V1low/RConn1 -- ADC Low1/LConn1 -- C1low_electrolytic/LConn1 -- C1low_ceramic/LConn1
  Switch3/LConn1 -- Controlled Current Source3/LConn1 -- Switch1/LConn1 -- Current Measurement/LConn1 -- Ideal Switch1/RConn1 -- Voltage Measurement/LConn1 -- Current Measurement1/RConn1 -- Ideal Switch2/RConn1 -- ADC High/LConn1 -- Controlled Current Source1/LConn1 -- Controlled Current Source2/LConn1
  VHigh_GND/RConn1 -- Voltage Measurement/LConn2 -- feeder VCC/RConn1 -- ADC High/RConn1 -- Chigh/RConn1 -- Controlled Current Source2/RConn1 -- Controlled Current Source3/RConn1 -- Switch2/RConn1 -- Low_GND/RConn1 -- v1Low/LConn2 -- ADC Low1/RConn1 -- Switch7/RConn1 -- C1low_ceramic/RConn1 -- v2Low/LConn2 -- ADC Low2/RConn1 -- Switch8/RConn1 -- C2low_ceramic/RConn1 -- Shottky2/LConn1 -- Switch4/RConn1 -- Shottky4/LConn1 -- Controlled Current Source1/RConn1 -- Meas Feeder/RConn1
  Current Measurement5/RConn1 -- v2Low/LConn1 -- ADC Low2/LConn1 -- C2low_electrolytic/LConn1 -- C2low_ceramic/LConn1
  Inductance2/RConn1 -- Switch4/LConn1 -- Switch3/RConn1 -- Shottky4/RConn1
  Switch1/RConn1 -- Inductance1/RConn1 -- Shottky2/RConn1 -- Switch2/LConn1
  Meas Feeder/LConn1 -- Ideal Switch1/LConn1
  Inductance2/LConn1 -- Current Measurement5/LConn1
  Switch7/LConn1 -- C1low_electrolytic/RConn1
  Ideal Switch2/LConn1 -- feeder VCC/LConn1
  Switch8/LConn1 -- C2low_electrolytic/RConn1
  Current Measurement/RConn1 -- Chigh/LConn1
  VHigh/RConn1 -- Current Measurement1/LConn1
  Current Measurement6/LConn1 -- Inductance1/LConn1
